simulink model "BEV_Thermal_Management"  (R2025a)
settings: Solver=ode23t  StartTime=0  StopTime=765  MaxStep=5  RelTol=1e-3  AbsTol=1e-3
model workspace: external: MATLAB File BEV_Thermal_Management_param.m (data not in the file)
undefined symbols (not defined in the file): Battery, bulb, cabin_doors_conductivity, cabin_duct_area, cabin_glass_conductivity, cabin_roof_conductivity, cabin_T_init, chiller_area_primary, chiller_N_baffles, chiller_N_tubes, chiller_tube_D, chiller_tube_L, chiller_wall_conductivity, chiller_wall_thickness, compressor_rpm_LUT, condenser_air_area_flow, condenser_air_area_primary, condenser_W, condenser_wall_conductivity, condenser_wall_thickness, coolant_channel_D, coolant_pipe_area, coolant_pipe_D, coolant_T_init, coolant_tank_area, coolant_tank_volume, coolant_valve_D_ratio_max, coolant_valve_D_ratio_min, coolant_valve_displacement, coolant_valve_S_max, cycle, DCDC, Edrive, evaporator_air_area_flow, evaporator_air_area_primary, evaporator_W, evaporator_wall_conductivity, evaporator_wall_thickness, heater_max_power, ModuleType1, outlet, ptc_max_power, pump_speed_max, radiationReflectionShields, radiator_air_area_flow, radiator_air_area_primary, radiator_W, radiator_wall_conductivity, radiator_wall_thickness, refrigerant_alpha_init, refrigerant_pipe_D, transRatio
libraries: fl_lib x264, nesl_utility x91, SimscapeFluids_lib x22, sdl_lib x13, ee_lib x9, nesl_utility_internal x4, slpidlib x3, BatteryProtection x3, batt_lib x2, BatteryCurrentManagement x1, autolibsharedcommon x1, simulink x1
(part 2 of 9)

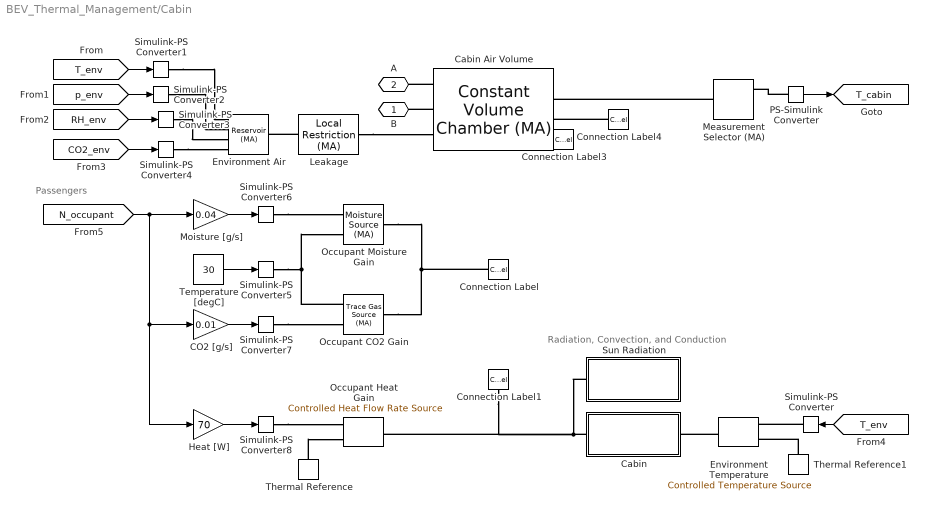
== system BEV_Thermal_Management/Cabin ==
  note: Radiation, Convection, and Conduction
  note: Passengers
  CO2 [g/s] : Gain  Gain=0.01
  Cabin : Subsystem  Tag=PublishSubsystem  mask(Cabin Heat Transfer){glass_area=3, glass_thickness=0.004, glass_mass=3 * 0.004 * 2600, glass_specific_heat=840, glass_conductivity=cabin_glass_conductivity, glass_heat_coeff=40, glass_initial_temperature=cabin_T_init, doors_area=4, doors_thickness=0.06, doors_mass=75, doors_specific_heat=500, doors_conductivity=cabin_doors_conductivity, doors_heat_coeff=40, doors_initial_temperature=cabin_T_init, roof_area=2, roof_thickness=0.04, roof_mass=30, roof_specific_heat=500, roof_conductivity=cabin_roof_conductivity, roof_heat_coeff=40, roof_initial_temperature=cabin_T_init}
      mask prompts: glass_area "Area (m^2)"; glass_thickness "Thickness (m)"; glass_mass "Mass (kg)"; glass_specific_heat "Specific heat (J/kg/K)"; glass_conductivity "Thermal conductivity (W/m/K)"; glass_heat_coeff "Convective heat transfer coefficient (W/m^2/K)"; glass_initial_temperature "Initial temperature (K)"; doors_area "Area (m^2)"; doors_thickness "Thickness (m)"; doors_mass "Mass (kg)"; doors_specific_heat "Specific heat (J/kg/K)"; doors_conductivity "Thermal conductivity (W/m/K)"; doors_heat_coeff "Convective heat transfer coefficient (W/m^2/K)"; doors_initial_temperature "Initial temperature (K)"; roof_area "Area (m^2)"; roof_thickness "Thickness (m)"; roof_mass "Mass (kg)"; roof_specific_heat "Specific heat (J/kg/K)"; roof_conductivity "Thermal conductivity (W/m/K)"; roof_heat_coeff "Convective heat transfer coefficient (W/m^2/K)"; roof_initial_temperature "Initial temperature (K)"
      mask DialogControl GlassTabVar Prompt: Glass
      mask DialogControl DoorsTabVar Prompt: Doors
      mask DialogControl RoofTabVar Prompt: Roof
  Cabin Air Volume : fl_lib/Moist Air/Elements/Constant Volume Chamber (MA)  volume=3 m^3  num_ports=foundation.enum.num_ports.three  area_A=cabin_duct_area m^2  area_B=cabin_duct_area m^2  area_C=1 m^2  area_D=0.01 m^2  RH_ws=1  time_constant_cond=1e-3 s  time_constant_evap=1e-3 s  fraction_entrained=1  moisture_trace_gas_source=foundation.enum.moisture_trace_gas_source.controlled  moisture_source_spec=foundation.enum.MoistureSourceSpec.WaterVapor  vapor_from_liquid=false  moisture_mass_flow=0 kg/s  moisture_temperature_spec=foundation.enum.temperature_spec.atmospheric  moisture_temperature=293.15 K  trace_gas_mass_flow=0 kg/s  trace_gas_temperature_spec=foundation.enum.temperature_spec.atmospheric  trace_gas_temperature=293.15 K  p_init=cabin_p_init MPa  p_init_priority=foundation.enum.Priority.High  T_init=cabin_T_init K  T_init_priority=foundation.enum.Priority.High  humidity_spec=foundation.enum.HumiditySpec.RelativeHumidity  RH_init=cabin_RH_init  RH_init_priority=foundation.enum.Priority.High  x_w_init=0  x_w_init_priority=foundation.enum.Priority.None  y_w_init=0  y_w_init_priority=foundation.enum.Priority.None  HR_init=0  HR_init_priority=foundation.enum.Priority.None  Tw_init=287 K  Tw_init_priority=foundation.enum.Priority.High  trace_gas_spec=foundation.enum.trace_gas_spec.mole_fraction  x_g_init=0  x_g_init_priority=foundation.enum.Priority.None  y_g_init=cabin_CO2_init  y_g_init_priority=foundation.enum.Priority.High  r_d_init=0  r_d_init_priority=foundation.enum.Priority.High
      settings: InternalSimscapePortConfiguration="{\"Bottom\":[],\"Left\":[{\"id\":\"A\",\"label\":\"A\",\"type\":\"foundation.moist_air.moist_air\"},{\"id\":\"B\",\"label\":\"B\",\"type\":\"foundation.moist_air.moist_air\"},{\"id\":\"C\",\"label\":\"C\",\"type\":\"foundation.moist_air.moist_air\"}],\"Right\":[{\"id\":\"W\",\"label\":\"W\",\"type\":\"output\"},{\"id\":\"F\",\"label\":\"F\",\"type\":\"output\"},{\"id\":\"H\",\"label\":\"H\",\"type\":\"foundation.thermal.thermal\"},{\"id\":\"S\",\"label\":\"S\",\"type\":\"foundation.moist_air.moist_air_source\"}],\"Top\":[]}"
  Connection Label : ConnectionLabel  Label=passenger_air
  Connection Label1 : ConnectionLabel  Label=int_and_ext_heat
  Connection Label3 : ConnectionLabel  Label=passenger_air
  Connection Label4 : ConnectionLabel  Label=int_and_ext_heat
  Environment Air : fl_lib/Moist Air/Elements/Reservoir (MA)  pressure_input=true  pressure_spec=foundation.enum.pressure_spec.atmospheric  reservoir_pressure=0.101325 MPa  temperature_input=true  temperature_spec=foundation.enum.temperature_spec.atmospheric  reservoir_temperature=293.15 K  humidity_input=true  humidity_spec=foundation.enum.HumiditySpec.RelativeHumidity  reservoir_RH=0.5  reservoir_x_w=0.01  reservoir_y_w=0.01  reservoir_HR=0.01  reservoir_Tw=287 K  trace_gas_input=true  trace_gas_spec=foundation.enum.trace_gas_spec.mole_fraction  reservoir_x_g=0.001  reservoir_y_g=0.001  water_droplets_input=false  reservoir_r_d=0  RH_ws=1  area_A=1 m^2  input_error_spec=foundation.enum.input_range_error.warn
      settings: InternalSimscapePortConfiguration="{\"Bottom\":[],\"Left\":[{\"id\":\"A\",\"label\":\"A\",\"type\":\"foundation.moist_air.moist_air\"}],\"Right\":[{\"id\":\"T\",\"label\":\"T\",\"type\":\"input\"},{\"id\":\"P\",\"label\":\"P\",\"type\":\"input\"},{\"id\":\"W\",\"label\":\"W\",\"type\":\"input\"},{\"id\":\"G\",\"label\":\"G\",\"type\":\"input\"}],\"Top\":[]}"
  Environment Temperature : fl_lib/Thermal/Thermal Sources/Controlled Temperature Source
  Heat [W] : Gain  Gain=70
  Leakage : fl_lib/Moist Air/Elements/Local Restriction (MA)  restriction_type=foundation.enum.restriction_type.fixed  restriction_area=0.004 m^2  min_area=1e-10 m^2  max_area=0.005 m^2  area=1 m^2  Cd=0.8  B_lam=0.999
      settings: InternalSimscapePortConfiguration="{\"Bottom\":[],\"Left\":[{\"id\":\"A\",\"label\":\"A\",\"type\":\"foundation.moist_air.moist_air\"}],\"Right\":[{\"id\":\"B\",\"label\":\"B\",\"type\":\"foundation.moist_air.moist_air\"}],\"Top\":[]}"
  Measurement Selector (MA) : fl_lib/Moist Air/Sensors/Measurement Selector (MA)  moisture_spec=foundation.enum.moisture_spec.relative_humidity  trace_gas_spec=foundation.enum.trace_gas_spec.mole_fraction
      settings: InternalSimscapePortConfiguration="{\"Bottom\":[],\"Left\":[{\"id\":\"F\",\"label\":\"F\",\"type\":\"input\"}],\"Right\":[{\"id\":\"P\",\"label\":\"P\",\"type\":\"output\"},{\"id\":\"T\",\"label\":\"T\",\"type\":\"output\"},{\"id\":\"W\",\"label\":\"W\",\"type\":\"output\"},{\"id\":\"G\",\"label\":\"G\",\"type\":\"output\"},{\"id\":\"D\",\"label\":\"D\",\"type\":\"output\"}],\"Top\":[]}"
  Moisture [g/s] : Gain  Gain=0.04
  Occupant CO2 Gain : fl_lib/Moist Air/Sources/Moisture & Trace Gas Sources/Trace Gas Source (MA)  source_type=foundation.enum.constant_controlled.controlled  trace_gas_mass_flow=0 kg/s  temperature_spec=foundation.enum.temperature_spec.atmospheric  trace_gas_temperature=293.15 K  Phi_S_specify=off  Phi_S_priority=None  Phi_S=0 kW  Phi_S_nominal_specify=off  Phi_S_nominal_value=1  Phi_S_nominal_unit=kW  mdot_g_S_specify=off  mdot_g_S_priority=None  mdot_g_S=0 kg/s  mdot_g_S_nominal_specify=off  mdot_g_S_nominal_value=1  mdot_g_S_nominal_unit=kg/s
      settings: InternalSimscapePortConfiguration="{\"Bottom\":[],\"Left\":[{\"id\":\"S\",\"label\":\"S\",\"type\":\"foundation.moist_air.moist_air_source\"}],\"Right\":[{\"id\":\"M\",\"label\":\"M\",\"type\":\"input\"},{\"id\":\"T\",\"label\":\"T\",\"type\":\"input\"}],\"Top\":[]}"
  Occupant Heat Gain : fl_lib/Thermal/Thermal Sources/Controlled Heat Flow Rate Source
  Occupant Moisture Gain : fl_lib/Moist Air/Sources/Moisture & Trace Gas Sources/Moisture Source (MA)  source_type=foundation.enum.constant_controlled.controlled  moisture_source_spec=foundation.enum.MoistureSourceSpec.WaterVapor  vapor_from_liquid=false  moisture_mass_flow=0 kg/s  temperature_spec=foundation.enum.temperature_spec.atmospheric  moisture_temperature=293.15 K  Phi_S_specify=off  Phi_S_priority=None  Phi_S=0 kW  Phi_S_nominal_specify=off  Phi_S_nominal_value=1  Phi_S_nominal_unit=kW  mdot_w_S_specify=off  mdot_w_S_priority=None  mdot_w_S=0 kg/s  mdot_w_S_nominal_specify=off  mdot_w_S_nominal_value=1  mdot_w_S_nominal_unit=kg/s  mdot_d_S_specify=off  mdot_d_S_priority=None  mdot_d_S=0 kg/s  mdot_d_S_nominal_specify=off  mdot_d_S_nominal_value=1  mdot_d_S_nominal_unit=kg/s
      settings: InternalSimscapePortConfiguration="{\"Bottom\":[],\"Left\":[{\"id\":\"S\",\"label\":\"S\",\"type\":\"foundation.moist_air.moist_air_source\"}],\"Right\":[{\"id\":\"M\",\"label\":\"M\",\"type\":\"input\"},{\"id\":\"T\",\"label\":\"T\",\"type\":\"input\"}],\"Top\":[]}"
  PS-Simulink Converter : nesl_utility/PS-Simulink Converter  PhysicalDomain=network_engine_domain  SubClassName=ps_output  LeftPortType=input  RightPortType=output  PseudoPeriodic=off  Frequencies=[]  VectorFormat=1-D array  Unit=degC  AffineConversion=on
  Simulink-PS Converter : nesl_utility/Simulink-PS Converter  PhysicalDomain=network_engine_domain  SubClassName=ps_input  LeftPortType=input  RightPortType=output  PseudoPeriodic=off  Frequencies=[]  NoiseDistribution=none  NoiseParameters=[]  Unit=degC  AffineConversion=on  FilteringAndDerivatives=provide  SimscapeFilterOrder=1  InputFilterTimeConstant=0.001  UdotUserProvided=0
  Simulink-PS Converter1 : nesl_utility/Simulink-PS Converter  PhysicalDomain=network_engine_domain  SubClassName=ps_input  LeftPortType=input  RightPortType=output  PseudoPeriodic=off  Frequencies=[]  NoiseDistribution=none  NoiseParameters=[]  Unit=degC  AffineConversion=on  FilteringAndDerivatives=provide  SimscapeFilterOrder=1  InputFilterTimeConstant=0.001  UdotUserProvided=0
  Simulink-PS Converter2 : nesl_utility/Simulink-PS Converter  PhysicalDomain=network_engine_domain  SubClassName=ps_input  LeftPortType=input  RightPortType=output  PseudoPeriodic=off  Frequencies=[]  NoiseDistribution=none  NoiseParameters=[]  Unit=MPa  AffineConversion=off  FilteringAndDerivatives=provide  SimscapeFilterOrder=1  InputFilterTimeConstant=0.001  UdotUserProvided=0
  Simulink-PS Converter3 : nesl_utility/Simulink-PS Converter  PhysicalDomain=network_engine_domain  SubClassName=ps_input  LeftPortType=input  RightPortType=output  PseudoPeriodic=off  Frequencies=[]  NoiseDistribution=none  NoiseParameters=[]  Unit=1  AffineConversion=off  FilteringAndDerivatives=provide  SimscapeFilterOrder=1  InputFilterTimeConstant=0.001  UdotUserProvided=0
  Simulink-PS Converter4 : nesl_utility/Simulink-PS Converter  PhysicalDomain=network_engine_domain  SubClassName=ps_input  LeftPortType=input  RightPortType=output  PseudoPeriodic=off  Frequencies=[]  NoiseDistribution=none  NoiseParameters=[]  Unit=1  AffineConversion=off  FilteringAndDerivatives=provide  SimscapeFilterOrder=1  InputFilterTimeConstant=0.001  UdotUserProvided=0
  Simulink-PS Converter5 : nesl_utility/Simulink-PS Converter  PhysicalDomain=network_engine_domain  SubClassName=ps_input  LeftPortType=input  RightPortType=output  PseudoPeriodic=off  Frequencies=[]  NoiseDistribution=none  NoiseParameters=[]  Unit=degC  AffineConversion=on  FilteringAndDerivatives=provide  SimscapeFilterOrder=1  InputFilterTimeConstant=0.001  UdotUserProvided=0
  Simulink-PS Converter6 : nesl_utility/Simulink-PS Converter  PhysicalDomain=network_engine_domain  SubClassName=ps_input  LeftPortType=input  RightPortType=output  PseudoPeriodic=off  Frequencies=[]  NoiseDistribution=none  NoiseParameters=[]  Unit=g/s  AffineConversion=off  FilteringAndDerivatives=provide  SimscapeFilterOrder=1  InputFilterTimeConstant=0.001  UdotUserProvided=0
  Simulink-PS Converter7 : nesl_utility/Simulink-PS Converter  PhysicalDomain=network_engine_domain  SubClassName=ps_input  LeftPortType=input  RightPortType=output  PseudoPeriodic=off  Frequencies=[]  NoiseDistribution=none  NoiseParameters=[]  Unit=g/s  AffineConversion=off  FilteringAndDerivatives=provide  SimscapeFilterOrder=1  InputFilterTimeConstant=0.001  UdotUserProvided=0
  Simulink-PS Converter8 : nesl_utility/Simulink-PS Converter  PhysicalDomain=network_engine_domain  SubClassName=ps_input  LeftPortType=input  RightPortType=output  PseudoPeriodic=off  Frequencies=[]  NoiseDistribution=none  NoiseParameters=[]  Unit=W  AffineConversion=off  FilteringAndDerivatives=provide  SimscapeFilterOrder=1  InputFilterTimeConstant=0.001  UdotUserProvided=0
  Sun Radiation : Subsystem
      mask Display: disp('Sun\nRadiation')
  Temperature [degC] : Constant  Value=30
  Thermal Reference : fl_lib/Thermal/Thermal Elements/Thermal Reference
  Thermal Reference1 : fl_lib/Thermal/Thermal Elements/Thermal Reference
  B : PMIOPort  Side=Left
  A : PMIOPort  Port=2  Side=Right
  tag scope: T_cabin=global
  wires:
  PS-Simulink Converter/1 -> [T_cabin]
  [T_env] -> Simulink-PS Converter1/1
  [p_env] -> Simulink-PS Converter2/1
  [RH_env] -> Simulink-PS Converter3/1
  [CO2_env] -> Simulink-PS Converter4/1
  [T_env] -> Simulink-PS Converter/1
  Moisture [g/s]/1 -> Simulink-PS Converter6/1
  CO2 [g/s]/1 -> Simulink-PS Converter7/1
  Heat [W]/1 -> Simulink-PS Converter8/1
  [N_occupant] -> Moisture [g/s]/1, Heat [W]/1, CO2 [g/s]/1
  Temperature [degC]/1 -> Simulink-PS Converter5/1
  connections:
  Cabin Air Volume/LConn1 -- A/RConn1
  Cabin Air Volume/LConn2 -- B/RConn1
  Simulink-PS Converter3/RConn1 -- Environment Air/RConn3
  Simulink-PS Converter4/RConn1 -- Environment Air/RConn4
  Simulink-PS Converter2/RConn1 -- Environment Air/RConn2
  Simulink-PS Converter1/RConn1 -- Environment Air/RConn1
  Leakage/RConn1 -- Environment Air/LConn1
  Leakage/LConn1 -- Cabin Air Volume/LConn3
  Occupant Moisture Gain/LConn1 -- Occupant CO2 Gain/LConn1 -- Connection Label/LConn1
  Sun Radiation/LConn1 -- Occupant Heat Gain/LConn1 -- Connection Label1/LConn1 -- Cabin/LConn1
  Thermal Reference/LConn1 -- Occupant Heat Gain/RConn2
  Simulink-PS Converter5/RConn1 -- Occupant CO2 Gain/RConn2 -- Occupant Moisture Gain/RConn2
  Simulink-PS Converter6/RConn1 -- Occupant Moisture Gain/RConn1
  Simulink-PS Converter7/RConn1 -- Occupant CO2 Gain/RConn1
  Simulink-PS Converter8/RConn1 -- Occupant Heat Gain/RConn1
  Environment Temperature/LConn1 -- Cabin/RConn1
  Thermal Reference1/LConn1 -- Environment Temperature/RConn2
  Simulink-PS Converter/RConn1 -- Environment Temperature/RConn1
  Measurement Selector (MA)/LConn1 -- Cabin Air Volume/RConn2
  PS-Simulink Converter/LConn1 -- Measurement Selector (MA)/RConn2
  Connection Label4/LConn1 -- Cabin Air Volume/RConn3
  Connection Label3/LConn1 -- Cabin Air Volume/RConn4

== system BEV_Thermal_Management/Charger ==
  note: 1 means that the vehicle is charging, otherwise 0
  Charger Model : Subsystem  Variant=on  VariantControlMode=label  LabelModeActiveChoice=no charger
  PWRS2 : Subsystem
      mask Display: disp(get_param(gcb,'Name'));
  A : PMIOPort  Side=Left
  HV : PMIOPort  Port=2  Side=Left
  B : PMIOPort  Port=3  Side=Right
  tag scope: BatChrgCrnt=global
  wires:
  [VCells] -> Charger Model/1(Voltage Cell)
  [chargingMode] -> Charger Model/2(Charging Logic)
  Charger Model/1(Battery Charging Current) -> [BatChrgCrnt]
  connections:
  A/RConn1 -- Charger Model/LConn1
  PWRS2/RConn1 -- HV/RConn1
  PWRS2/LConn1 -- Charger Model/RConn1
  B/RConn1 -- Charger Model/RConn2

== system BEV_Thermal_Management/Chiller ==
  note: The chiller is assumed to be a shell-and-tube type heat exchanger that lets the refrigerant absorb heat from the coolant.
      | This way the coolant (water glycol) form the battery is cooled and heats the refrigerant (R 123)
  Chiller : SimscapeFluids_lib/Heat Exchangers/Two-Phase Fluid - Thermal Liquid/Condenser Evaporator (TL-2P)  flow_arrangement=fluids.heat_exchangers.enum.FlowArrangementTL2P.Cross  cross_flow_arrangement=fluids.heat_exchangers.enum.CrossFlowArrangementTL2P.UnmixedMixed  R_wall=chiller_wall_thickness / chiller_area_primary / chiller_wall_conductivity K/W  wall_thermal_mass=false  mass_wall=1 kg  cp_wall=490 J/(K*kg)  area_A1=coolant_pipe_area m^2  area_B1=coolant_pipe_area m^2  area_A2=pi * refrigerant_pipe_D^2 / 4 m^2  area_B2=pi * refrigerant_pipe_D^2 / 4 m^2  flow_geometry_TL=fluids.heat_exchangers.enum.FlowGeometryTL.AcrossTubeBank  tube_num_TL=1  tube_length_TL=5 m  tube_cross_section_TL=fluids.heat_exchangers.enum.TubeCrossSection.Circular  tube_diameter_TL=0.1 m  tube_width_TL=0.1 m  tube_height_TL=0.1 m  tube_inner_diameter_TL=0.05 m  tube_outer_diameter_TL=0.1 m  tube_flow_area_TL=0.01 m^2  tube_wetted_perimeter_TL=0.4 m  tube_heat_perimeter_TL=0.4 m  tube_pressure_loss_spec_TL=fluids.heat_exchangers.enum.TubePressureLossSpec.Haaland  tube_loss_coeff_TL=10  tube_local_pressure_loss_spec_TL=fluids.heat_exchangers.enum.LocalLossSpec.AggregateLength  tube_length_add_TL=0.1 m  tube_local_loss_coefficient_TL=0.1  tube_roughness_pressure_TL=15e-6 m  tube_Re_lam_pressure_TL=2000  tube_Re_tur_pressure_TL=4000  tube_shape_factor_generic_TL=64  tube_heat_coeff_spec_TL=fluids.heat_exchangers.enum.TubeHeatCoeffSpec.Gneilinski  tube_colburn_coeff_TL=[.023, .8, .33]  tube_roughness_heat_TL=15e-6 m  tube_Re_lam_heat_TL=2000  tube_Re_tur_heat_TL=4000  tube_Nu_lam_generic_TL=3.66  bank_arrangement_TL=fluids.heat_exchangers.enum.BankArrangement.Staggered  bank_num_rows_TL=sqrt(chiller_N_tubes) * (chiller_N_baffles + 1)  bank_tubes_per_row_TL=sqrt(chiller_N_tubes)  bank_width_TL=chiller_tube_L / (chiller_N_baffles + 1) m  bank_tube_diameter_TL=chiller_tube_D m  bank_longitudinal_pitch_TL=2 * chiller_tube_D m  bank_transverse_pitch_TL=2 * chiller_tube_D m  bank_pressure_loss_spec_TL=fluids.heat_exchangers.enum.BankPressureLossSpec.Martin  bank_euler_TL=10  bank_heat_coeff_spec_TL=fluids.heat_exchangers.enum.BankHeatCoeffSpec.Martin  bank_colburn_coeff_TL=[.27, .63, .36]  generic_flow_area_TL=0.01 m^2  generic_heat_area_TL=2 m^2  generic_volume_TL=0.05 m^3  generic_loss_coeff_TL=10  generic_colburn_coeff_TL=[.023, .8, .33]  fouling_factor_TL=0.1 m^2*K/kW  fin_area_TL=chiller_area_baffles m^2  fin_efficiency_TL=0.5  p_init_TL=coolant_p_init MPa  T_init_TL=coolant_T_init K  tube_num_2P=chiller_N_tubes  tube_length_2P=chiller_tube_L m  tube_cross_section_2P=fluids.heat_exchangers.enum.TubeCrossSection.Circular  tube_diameter_2P=chiller_tube_D m  tube_width_2P=0.1 m  tube_height_2P=0.1 m  tube_inner_diameter_2P=0.05 m  tube_outer_diameter_2P=0.1 m  tube_flow_area_2P=0.01 m^2  tube_wetted_perimeter_2P=0.4 m  tube_heat_perimeter_2P=0.4 m  tube_pressure_loss_spec_2P=fluids.heat_exchangers.enum.TubePressureLossSpec2P.Haaland  tube_loss_coeff_2P=10  tube_local_pressure_loss_spec_2P=fluids.heat_exchangers.enum.LocalLossSpec.AggregateLength  tube_length_add_2P=chiller_tube_Leq m  tube_local_loss_coefficient_2P=0.1  tube_roughness_pressure_2P=15e-6 m  tube_Re_lam_pressure_2P=2000  tube_Re_tur_pressure_2P=4000  tube_shape_factor_generic_2P=64  tube_heat_coeff_spec_2P=fluids.heat_exchangers.enum.TubeHeatCoeffSpec2P.GneilinskiCavalliniZecchin  tube_colburn_coeff_liq_2P=[.023, .8, .33]  tube_colburn_coeff_mix_2P=[.05, .8, .33]  tube_colburn_coeff_vap_2P=[.023, .8, .33]  tube_roughness_heat_2P=15e-6 m  tube_Re_lam_heat_2P=2000  tube_Re_tur_heat_2P=4000  tube_Nu_lam_generic_2P=3.66  fouling_factor_2P=0.1 m^2*K/kW  fin_area_2P=0 m^2  fin_efficiency_2P=0  energy_spec_2P=foundation.enum.energy_spec.void_fraction  p_init_2P=refrigerant_p_init MPa  T_init_2P=293.15 K  x_init_2P=0.5  alpha_init_2P=refrigerant_alpha_init  h_init_2P=1500 kJ/kg  u_init_2P=1500 kJ/kg
      settings: InternalSimscapePortConfiguration="{\"Bottom\":[],\"Left\":[{\"id\":\"A1\",\"label\":\"A1\",\"type\":\"foundation.thermal_liquid.thermal_liquid\"},{\"id\":\"B1\",\"label\":\"B1\",\"type\":\"foundation.thermal_liquid.thermal_liquid\"}],\"Right\":[{\"id\":\"A2\",\"label\":\"A2\",\"type\":\"foundation.two_phase_fluid.two_phase_fluid\"},{\"id\":\"B2\",\"label\":\"B2\",\"type\":\"foundation.two_phase_fluid.two_phase_fluid\"}],\"Top\":[{\"id\":\"Z\",\"label\":\"Z\",\"type\":\"output\"}]}"
  Flow Resistance (2P) : fl_lib/Two-Phase Fluid/Elements/Flow Resistance (2P)  delta_p_nominal=1e-4 MPa  mdot_nominal=0.01 kg/s  v_nominal=0 m^3/kg  area=pi * refrigerant_pipe_D^2 / 4 m^2  laminar_fraction=1e-3
      settings: InternalSimscapePortConfiguration="{\"Bottom\":[],\"Left\":[{\"id\":\"A\",\"label\":\"A\",\"type\":\"foundation.two_phase_fluid.two_phase_fluid\"}],\"Right\":[{\"id\":\"B\",\"label\":\"B\",\"type\":\"foundation.two_phase_fluid.two_phase_fluid\"}],\"Top\":[]}"
  SC7 : Subsystem
      mask Display: disp(get_param(gcb, 'Name'))
  SC8 : Subsystem
      mask Display: disp(get_param(gcb, 'Name'))
  SR3 : Subsystem
      mask Display: disp(get_param(gcb, 'Name'))
  SR4 : Subsystem
      mask Display: disp(get_param(gcb, 'Name'))
  Simscape Bus : SimscapeBus  HierarchyStrings=bulb;outlet
  B : PMIOPort  Side=Left
  A : PMIOPort  Port=2  Side=Right
  C : PMIOPort  Port=3  Side=Left
  D : PMIOPort  Port=4  Side=Right
  connections:
  SC7/RConn1 -- C/RConn1
  SC8/LConn1 -- D/RConn1
  Chiller/RConn1 -- SR3/LConn1
  SR4/RConn1 -- Chiller/RConn2 -- Simscape Bus/LConn1
  Simscape Bus/LConn2 -- SR3/RConn1
  A/RConn1 -- Simscape Bus/RConn1
  B/RConn1 -- Flow Resistance (2P)/RConn1
  Flow Resistance (2P)/LConn1 -- SR4/LConn1
  Chiller/LConn2 -- SC7/LConn1
  Chiller/LConn1 -- SC8/RConn1

== system BEV_Thermal_Management/Chiller Bypass Valve ==
  note: if it is equal to 1, the chiller is bypassed
  note: The chiller operates in an on-off manner depending on the battery temperature. This is controlled by the 3-way valve that either sends coolant to the chiller or bypasses the chiller.
  Bias : Bias  Bias=-1  SaturateOnIntegerOverflow=off
  Chiller Bypass Valve : SimscapeFluids_lib/Thermal Liquid/Valves & Orifices/Directional Control Valves/3-Way Directional Valve (TL)  open_orifices_pos=fluids.thermal_liquid.valves.directional_control_valves.enum.OpenOrifices3Way.PA  open_orifices_neg=fluids.thermal_liquid.valves.directional_control_valves.enum.OpenOrifices3Way.AT  area_spec=fluids.thermal_liquid.valves.directional_control_valves.enum.area_spec.identical  valve_spec=fluids.thermal_liquid.valves.enum.orifice_spec.linear  del_S_max=coolant_valve_displacement m  area_max=pi * (coolant_valve_D_ratio_max*coolant_pipe_D)^2 / 4 m^2  del_S_TLU=[0 0.002 0.004 0.007 0.017] m  valve_area_TLU=[1e-09, 2.0352e-07, 4.0736e-05, .00011438, .00034356] m^2  del_S_flow_TLU=[0 0.002 0.004 0.007 0.017] m  p_diff_TLU=[-.1, .3, .5, .7] MPa  vol_flow_TLU=1e-3 * [1.7e-05, 2e-05, 2.6e-05; .0035, .0045, .0053; .7, .9, 1.06; 1.96, 2.5, 3; 6, 7.7, 9.13] m^3/s  mdot_TLU=[-1e-05, 1.7e-05, 2e-05, 2.6e-05; -.002, .0035, .0045, .0053; -.4, .7, .9, 1.06; -1.13, 1.96, 2.5, 3; -3.45, 6, 7.7, 9.13] kg/s  T_ref_in=293.15 K  p_ref_in=0.101325 MPa  area_leak=pi * (coolant_valve_D_ratio_min*coolant_pipe_D)^2 / 4 m^2  Cd=0.7  Re_c=12  smoothing_factor=0.01  pressure_recovery=simscape.enum.onoff.on  area=coolant_pipe_area m^2  S_max_PA=coolant_valve_S_max m  del_S_max_PA=coolant_valve_displacement-(coolant_valve_displacement)*(pi * (coolant_valve_D_ratio_min*coolant_pipe_D)^2 / 4)/(pi * (coolant_valve_D_ratio_max*coolant_pipe_D)^2 / 4) m  area_max_PA=pi * (coolant_valve_D_ratio_max*coolant_pipe_D)^2 / 4 m^2  del_S_TLU_PA=[0 0.002 0.004 0.007 0.017] m  valve_area_TLU_PA=[1e-09, 2.0352e-07, 4.0736e-05, .00011438, .00034356] m^2  del_S_flow_TLU_PA=[0 0.002 0.004 0.007 0.017] m  p_diff_TLU_PA=[-.1, .3, .5, .7] MPa  vol_flow_TLU_PA=1e-3 * [1.7e-05, 2e-05, 2.6e-05; .0035, .0045, .0053; .7, .9, 1.06; 1.96, 2.5, 3; 6, 7.7, 9.13] m^3/s  mdot_TLU_PA=[-1e-05, 1.7e-05, 2e-05, 2.6e-05; -.002, .0035, .0045, .0053; -.4, .7, .9, 1.06; -1.13, 1.96, 2.5, 3; -3.45, 6, 7.7, 9.13] kg/s  S_max_AT=-coolant_valve_S_max m  del_S_max_AT=coolant_valve_displacement-(coolant_valve_displacement)*(pi * (coolant_valve_D_ratio_min*coolant_pipe_D)^2 / 4)/(pi * (coolant_valve_D_ratio_max*coolant_pipe_D)^2 / 4) m  area_max_AT=pi * (coolant_valve_D_ratio_max*coolant_pipe_D)^2 / 4 m^2  del_S_TLU_AT=[0 0.002 0.004 0.007 0.017] m  valve_area_TLU_AT=[1e-09, 2.0352e-07, 4.0736e-05, .00011438, .00034356] m^2  del_S_flow_TLU_AT=[0 0.002 0.004 0.007 0.017] m  p_diff_TLU_AT=[-.1, .3, .5, .7] MPa  vol_flow_TLU_AT=1e-3 * [1.7e-05, 2e-05, 2.6e-05; .0035, .0045, .0053; .7, .9, 1.06; 1.96, 2.5, 3; 6, 7.7, 9.13] m^3/s  mdot_TLU_AT=[-1e-05, 1.7e-05, 2e-05, 2.6e-05; -.002, .0035, .0045, .0053; -.4, .7, .9, 1.06; -1.13, 1.96, 2.5, 3; -3.45, 6, 7.7, 9.13] kg/s  S_max_PT=2.5e-3 m  del_S_max_PT=0.005 m  area_max_PT=1e-4 m^2  del_S_TLU_PT=[0, .002, .004, .007, .017] m  valve_area_TLU_PT=[1e-09, 2.0352e-07, 4.0736e-05, .00011438, .00034356] m^2  del_S_flow_TLU_PT=[0, .002, .004, .007, .017] m  p_diff_TLU_PT=[.3, .5, .7] MPa  vol_flow_TLU_PT=1e-3 * [1.7e-05, 2e-05, 2.6e-05; .0035, .0045, .0053; .7, .9, 1.06; 1.96, 2.5, 3; 6, 7.7, 9.13] m^3/s  mdot_TLU_PT=[1.7e-05, 2e-05, 2.6e-05; .0035, .0045, .0053; .7, .9, 1.06; 1.96, 2.5, 3; 6, 7.7, 9.13] kg/s
      settings: InternalSimscapePortConfiguration="{\"Bottom\":[],\"Left\":[{\"id\":\"A\",\"label\":\"A\",\"type\":\"foundation.thermal_liquid.thermal_liquid\"}],\"Right\":[{\"id\":\"S\",\"label\":\"S\",\"type\":\"input\"},{\"id\":\"P\",\"label\":\"P\",\"type\":\"foundation.thermal_liquid.thermal_liquid\"},{\"id\":\"T\",\"label\":\"T\",\"type\":\"foundation.thermal_liquid.thermal_liquid\"}],\"Top\":[]}"
  Flow Resistance (TL) : fl_lib/Thermal Liquid/Elements/Flow Resistance (TL)  delta_p_nominal=0.001 MPa  mdot_nominal=0.3 kg/s  area=coolant_pipe_area m^2  laminar_fraction=1e-3
  Gain : Gain  Gain=2
  Max Valve Displacement [m] : Gain  Gain=coolant_valve_displacement
  Simulink-PS Converter : nesl_utility/Simulink-PS Converter  PhysicalDomain=network_engine_domain  SubClassName=ps_input  LeftPortType=input  RightPortType=output  PseudoPeriodic=off  Frequencies=[]  NoiseDistribution=none  NoiseParameters=[]  Unit=m  AffineConversion=off  FilteringAndDerivatives=provide  SimscapeFilterOrder=1  InputFilterTimeConstant=0.001  UdotUserProvided=0
  Transfer Fcn : TransferFcn  Denominator=[1 1]
  A : PMIOPort  Side=Left
  C : PMIOPort  Port=2  Side=Left
  B : PMIOPort  Port=3  Side=Right
  wires:
  Max Valve Displacement [m]/1 -> Simulink-PS Converter/1
  Bias/1 -> Max Valve Displacement [m]/1
  Gain/1 -> Bias/1
  Transfer Fcn/1 -> Gain/1
  [cmd_chiller_bypass] -> Transfer Fcn/1
  connections:
  Chiller Bypass Valve/LConn1 -- A/RConn1
  Chiller Bypass Valve/RConn3 -- C/RConn1
  Chiller Bypass Valve/RConn1 -- Simulink-PS Converter/RConn1
  Chiller Bypass Valve/RConn2 -- Flow Resistance (TL)/LConn1
  Flow Resistance (TL)/RConn1 -- B/RConn1

== system BEV_Thermal_Management/Chiller Expansion Valve ==
  Chiller Expansion Valve : SimscapeFluids_lib/Two-Phase Fluid/Valves & Orifices/Flow Control Valves/Thermostatic Expansion Valve (2P)  valve_parameterization=fluids.two_phase_fluid.valves_orifices.flow_control_valves.enum.ThermostaticExpansionValveParameterization.Nominal  capacity_spec=fluids.two_phase_fluid.valves_orifices.flow_control_valves.enum.ThermostaticExpansionValveCapacitySpec.HeatTransfer  Q_nominal=4500 W  Q_max=7000 W  mdot_nominal=0.005 kg/s  mdot_max=0.008 kg/s  pressure_spec=fluids.two_phase_fluid.valves_orifices.flow_control_valves.enum.ThermostaticExpansionValvePressureSpec.SaturationTemperature  p_cond_nominal=1.5 MPa  p_evap_nominal=0.5 MPa  T_cond_nominal=40 degC  T_evap_nominal=1 degC  delta_T_sub=5 deltaK  delta_T_nominal=10 deltaK  delta_T_static=5 deltaK  mop=fluids.two_phase_fluid.valves_orifices.flow_control_valves.enum.ThermostaticExpansionValveMOP.Off  p_mop=0.5 MPa  T_mop=288.15 K  T_evap_out_TLU1=0 : 10 : 40 degC  p_bulb_TLU1=0.3 : 0.1 : 0.7 MPa  lift_TLU2=0 : 0.15 : 0.6 mm  p_evap_TLU2=0.3 : -0.05 : 0.1 MPa  lift_TLU3=0 : 0.15 : 0.6 mm  mdot_TLU3=0 : 0.015 : 0.06 kg/s  p_cond_ref=2 MPa  p_evap_ref=0.2 MPa  T_evap_out_ref=0 degC  delta_T_sub_ref=5 deltaK  pressure_equalization=fluids.two_phase_fluid.valves_orifices.flow_control_valves.enum.ThermostaticExpansionValveEqualization.External  bulb_dynamics=simscape.enum.onoff.off  tau_bulb=20 s  leakage_fraction=1e-6  smoothing_factor=0.01  B_lam=0.999  tau_x=0.1 s  area=pi * refrigerant_pipe_D^2 / 4 m^2
      settings: InternalSimscapePortConfiguration="{\"Bottom\":[],\"Left\":[{\"id\":\"A\",\"label\":\"A\",\"type\":\"foundation.two_phase_fluid.two_phase_fluid\"}],\"Right\":[{\"id\":\"B\",\"label\":\"B\",\"type\":\"foundation.two_phase_fluid.two_phase_fluid\"}],\"Top\":[{\"id\":\"S\",\"label\":\"S\",\"type\":\"foundation.two_phase_fluid.two_phase_fluid\"},{\"id\":\"E\",\"label\":\"E\",\"type\":\"foundation.two_phase_fluid.two_phase_fluid\"}]}"
  Simscape Bus : SimscapeBus  HierarchyStrings=bulb;outlet
  B : PMIOPort  Side=Left
  A : PMIOPort  Port=2  Side=Right
  connections:
  A/RConn1 -- Chiller Expansion Valve/LConn1
  Simscape Bus/LConn2 -- Chiller Expansion Valve/RConn1
  Chiller Expansion Valve/LConn3 -- Chiller Expansion Valve/LConn2 -- Simscape Bus/LConn1
  Simscape Bus/RConn1 -- B/RConn1

== system BEV_Thermal_Management/Compressor ==
  note: Electrical Power Demand
  note: Command
  note: Compressor Model
  note: The compressor drives the flow in the refrigerant loop. It is controlled to maintain a pressure of 0.3 MPa in the chiller and the evaporator, which corresponds to a saturation temperature of around 1 degC.
      |
      | The power required by the compressor is calculatred and attached to the battery circuit
  Battery voltage : fl_lib/Electrical/Electrical Sensors/Voltage Sensor
  Controlled Current Source : fl_lib/Electrical/Electrical Sources/Controlled Current Source
  Electrical Reference : fl_lib/Electrical/Electrical Elements/Electrical Reference
  Electrical Reference1 : fl_lib/Electrical/Electrical Elements/Electrical Reference
  Ideal Angular Velocity Source : fl_lib/Mechanical/Mechanical Sources/Ideal Angular Velocity Source
  Max Speed [rpm] : Gain  Gain=max(compressor_rpm_LUT)
  Mechanical Rotational Reference : fl_lib/Mechanical/Rotational Elements/Mechanical Rotational Reference
  PS-Simulink Converter2 : nesl_utility/PS-Simulink Converter  PhysicalDomain=network_engine_domain  SubClassName=ps_output  LeftPortType=input  RightPortType=output  PseudoPeriodic=off  Frequencies=[]  VectorFormat=inherit  Unit=degC  AffineConversion=off
  Positive-Displacement Compressor (2P) : SimscapeFluids_lib/Two-Phase Fluid/Fluid Machines/Positive-Displacement Compressor (2P)  dispSpec=fluids.two_phase_fluid.fluid_machines.enum.DisplacementSpecification.Displacement  v_disp=compressor_displacement cm^3/rev  mdot_nom=0.01 kg/s  omega_nom=1000 rpm  efficiencySpec=fluids.two_phase_fluid.fluid_machines.enum.VolumetricEfficiencyParameterization.Analytical  thermodynamicModelSpec=fluids.two_phase_fluid.fluid_machines.enum.ThermodynamicModel.Isentropic  n=1.2  eta_isen=0.65  eta_isen_TLU=[.95, .9, .85, .8, .75; .925, .875, .825, .775, .725; .875, .825, .775, .725, .675; .75, .7, .65, .6, .55]  eta_vol_nom=0.9  pr_TLU=[2, 4, 6, 8]  omega_TLU=[800, 1500, 2800, 3300, 4000] rpm  eta_vol_TLU=[.95, .9, .85, .8, .75; .925, .875, .825, .775, .725; .875, .825, .775, .725, .675; .75, .7, .65, .6, .55]  nominalSpec=fluids.two_phase_fluid.fluid_machines.enum.NominalConditionsSpecification.Pressure  pr_nom=4.6  p_in_nom=0.3 MPa  T_in_nom=11 degC  T_evap_nom=373.15 K  T_cond_nom=398.15 K  delta_T_nom=10 deltaK  mechanical_efficiency=0.95  area_A=pi * refrigerant_pipe_D^2 / 4 m^2  area_B=pi * refrigerant_pipe_D^2 / 4 m^2  VaporCheck=simscape.enum.assert.action.none
      settings: InternalSimscapePortConfiguration="{\"Bottom\":[],\"Left\":[{\"id\":\"A\",\"label\":\"A\",\"type\":\"foundation.two_phase_fluid.two_phase_fluid\"},{\"id\":\"C\",\"label\":\"C\",\"type\":\"foundation.mechanical.rotational.rotational\"}],\"Right\":[{\"id\":\"B\",\"label\":\"B\",\"type\":\"foundation.two_phase_fluid.two_phase_fluid\"},{\"id\":\"R\",\"label\":\"R\",\"type\":\"foundation.mechanical.rotational.rotational\"}],\"Top\":[]}"
  Power sensor : Subsystem
      settings: PortSchema="{\"entries\":[{\"content\":{\"sides\":[{\"content\":{\"connectorIds\":[\"LConn1\"]},\"type\":\"ConnectorPlacement.EquallySpacedRectSide\",\"uuid\":\"14aacb84-4d2c-4fe3-9667-966fc9affdc2\"},{\"content\":{\"connectorIds\":[\"RConn1\"],\"side\":\"RIGHT\"},\"type\":\"ConnectorPlacement.EquallySpacedRectSide\",\"uuid\":\"5f04cc75-bf75-44ff-ad13-d2b18990cf19\"},{\"content\":{\"connectorIds\":[\"LConn2\"],\"side\":\"TOP\"},\"type\":\"ConnectorPlacement.EquallySpacedRectSide\",\"uuid\":\"fdf9b4dd-6b03-4f92-a45a-c9cb867bd95a\"}]},\"type\":\"ConnectorPlacement.EquallySpacedConnector\",\"uuid\":\"3effddba-6f65-4497-8868-e18a0983ff0c\"}],\"packageUris\":[\"http://schema.mathworks.com/mf0/Connector/R2020b\"],\"version\":\"1.0\"}"
  Required current : fl_lib/Physical Signals/Functions/PS Divide
  Simulink-PS Converter : nesl_utility/Simulink-PS Converter  PhysicalDomain=network_engine_domain  SubClassName=ps_input  LeftPortType=input  RightPortType=output  PseudoPeriodic=off  Frequencies=[]  NoiseDistribution=none  NoiseParameters=[]  Unit=rpm  AffineConversion=off  FilteringAndDerivatives=provide  SimscapeFilterOrder=1  InputFilterTimeConstant=0.001  UdotUserProvided=0
  Terminator : Terminator
  Thermodynamic Properties Sensor (2P) : fl_lib/Two-Phase Fluid/Sensors/Thermodynamic Properties Sensor (2P)  temperature=true  enthalpy=false  density=false  specific_volume=false  entropy=false
      settings: InternalSimscapePortConfiguration="{\"Bottom\":[],\"Left\":[{\"id\":\"A\",\"label\":\"A\",\"type\":\"foundation.two_phase_fluid.two_phase_fluid\"}],\"Right\":[{\"id\":\"T\",\"label\":\"T\",\"type\":\"output\"}],\"Top\":[]}"
  Transfer Fcn : TransferFcn  Denominator=[0.5 1]
  B : PMIOPort  Side=Left
  A : PMIOPort  Port=2  Side=Right
  HV : PMIOPort  Port=3  Side=Right
  wires:
  Max Speed [rpm]/1 -> Simulink-PS Converter/1
  Transfer Fcn/1 -> Max Speed [rpm]/1
  [cmd_comp] -> Transfer Fcn/1
  PS-Simulink Converter2/1 -> Terminator/1  "tempRefCmpOut"
  connections:
  Battery voltage/LConn1 -- Controlled Current Source/RConn2 -- HV/RConn1
  Required current/RConn1 -- Controlled Current Source/RConn1
  Electrical Reference1/LConn1 -- Controlled Current Source/LConn1
  Battery voltage/RConn1 -- Required current/LConn2
  Electrical Reference/LConn1 -- Battery voltage/RConn2
  B/RConn1 -- Thermodynamic Properties Sensor (2P)/LConn1 -- Positive-Displacement Compressor (2P)/RConn1
  Mechanical Rotational Reference/LConn1 -- Positive-Displacement Compressor (2P)/LConn2 -- Ideal Angular Velocity Source/RConn2
  A/RConn1 -- Positive-Displacement Compressor (2P)/LConn1
  Simulink-PS Converter/RConn1 -- Ideal Angular Velocity Source/RConn1
  Power sensor/LConn1 -- Ideal Angular Velocity Source/LConn1
  Positive-Displacement Compressor (2P)/RConn2 -- Power sensor/RConn1
  Power sensor/LConn2 -- Required current/LConn1
  PS-Simulink Converter2/LConn1 -- Thermodynamic Properties Sensor (2P)/RConn1
